simulink model "DCHR_Dispatch_Stateflow_v14"  (R2026a)
settings: Solver=FixedStepDiscrete  StopTime=24  FixedStep=1
settings Model: Creator=Lysda  LastModifiedBy=Lysda

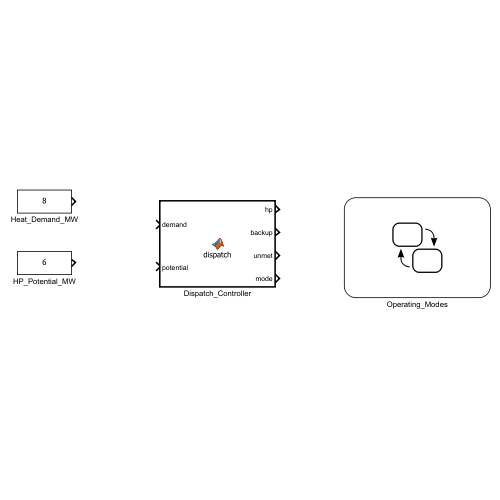
[thumbnail: Simulink's stored preview of the top-level diagram]
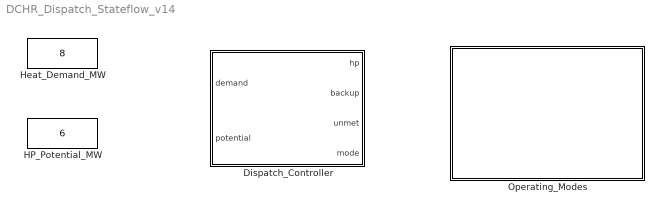
== system DCHR_Dispatch_Stateflow_v14 ==
  Dispatch_Controller : MATLAB Function  TreatAsAtomicUnit=on
  HP_Potential_MW : Constant  Value=6
  Heat_Demand_MW : Constant  Value=8
  Operating_Modes : Stateflow chart  TreatAsAtomicUnit=on

== matlab function DCHR_Dispatch_Stateflow_v14/Dispatch_Controller ==
  data: demand input; hp output; potential input; backup output; unmet output; mode output
function [hp,backup,unmet,mode] = dispatch(demand,potential)
%#codegen
hp=min(max(potential,0),max(demand,0));
backup=min(2,max(0,demand-hp));
unmet=max(0,demand-hp-backup);
mode=double(unmet>0)*2+double(unmet==0 && backup>0);
end

== stateflow chart DCHR_Dispatch_Stateflow_v14/Operating_Modes ==
  state RECOVERY
  state BACKUP
  (default) -> RECOVERY
  BACKUP -> RECOVERY : [false]
  RECOVERY -> BACKUP : [true]
